simulink model "TotemPoleBoostPFCConverter"  (R2026a)
settings: Solver=ode3  StopTime=0.05  MaxStep=1e-5  AbsTol=1e-3
PreLoadFcn:
  | TotemPoleBoostPFCDefaultInputParameters;
model workspace (MAT data in the model file):
  ConverterKey = "TotemPoleBoostPFC"
undefined symbols (not defined in the file): Rload_R, totemPoleDesign, Vref
libraries: ee_lib x27, nesl_utility x23, fl_lib x12, ConverterLibrary x1
(part 1 of 3)
settings Model: Creator=vsolaise  LastModifiedBy=vsolaise
settings SimscapeCC: SimscapeNominalValues="[{\"value\":\"1\",\"unit\":\"A\"},{\"value\":\"1\",\"unit\":\"bar\"},{\"value\":\"1\",\"unit\":\"cm^2\"},{\"value\":\"1\",\"unit\":\"cm^3/s\"},{\"value\":\"1\",\"unit\":\"kJ/kg\"},{\"value\":\"1\",\"unit\":\"kW\"},{\"value\":\"1\",\"unit\":\"l\"},{\"value\":\"1\",\"unit\":\"N\"},{\"value\":\"1\",\"unit\":\"N*m\"},{\"value\":\"1\",\"unit\":\"V\"}]"  SimscapeLogDecimation=12.0  SimscapeLogDataHistory=50000.0

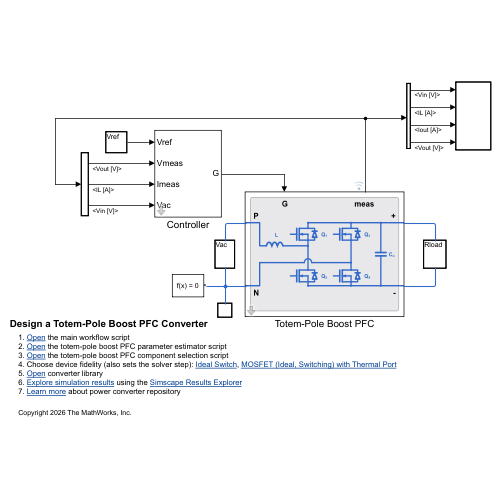
[thumbnail: Simulink's stored preview of the top-level diagram]
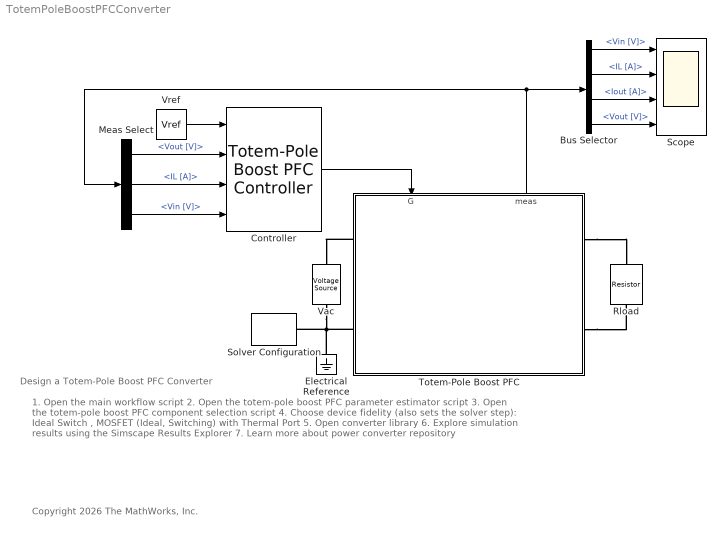
== system TotemPoleBoostPFCConverter ==
  note: Design a Totem-Pole Boost PFC Converter
  note: 1. Open the main workflow script
      | 2. Open the totem-pole boost PFC parameter estimator script
      | 3. Open the totem-pole boost PFC component selection script
      | 4. Choose device fidelity (also sets the solver step): Ideal Switch , MOSFET (Ideal, Switching) with Thermal Port
      | 5. Open converter library
      | 6. Explore simulation results using the Simscape Results Explorer
      | 7. Learn more about power converter repository
  note: Copyright 2026 The MathWorks, Inc.
  Bus Selector : BusSelector  OutputSignals=Vin [V],IL [A],Iout [A],Vout [V]
  Controller : ConverterLibrary/Controller/Power Factor Correction Converters/Totem-Pole Boost PFC Controller  outputSelect=PWM Signal  cntrlSelect=PI controller (Discrete)  VacRMS=totemPoleDesign.nomInputVoltage.value  VbaseDC=totemPoleDesign.outputVoltage.value  Pbase=totemPoleDesign.ratedPower.value  Fsw=totemPoleDesign.switchingFrequency.value  Fline=totemPoleDesign.lineFrequency.value  fastLegDeadTime=totemPoleController.fastLegDeadTime  slowLegTurnOnDelay=totemPoleController.slowLegTurnOnDelay  PrefPu=totemPoleController.PrefPu  iRefPeakMaxPu=totemPoleController.iRefPeakMaxPu  gateVoltageOn=totemPoleController.gateVoltageOn  gateVoltageOff=totemPoleController.gateVoltageOff  KpVoltage=totemPoleController.KpVoltage  KiVoltage=totemPoleController.KiVoltage  TsVoltage=totemPoleController.TsVoltage  KpCurrent=totemPoleController.KpCurrent  KiCurrent=totemPoleController.KiCurrent  dutyMax=totemPoleController.dutyMax  dutyMin=totemPoleController.dutyMin  TsCurrent=totemPoleController.TsCurrent
      link override Current Controller: LabelModeActiveChoice=PIDiscrete
      link override Gate Logic/Slow Leg Complementary PWM/Ramp Mode: LabelModeActiveChoice=FixedStep
      link override Output Mode: LabelModeActiveChoice=PWMSignal
      link override Output Mode/PWMSignal/Half Bridge PWM Generator/Ramp Mode: LabelModeActiveChoice=FixedStep
      link override Voltage Controller: LabelModeActiveChoice=PIDiscrete
      settings: SourceProductName=Simscape Power Converter Components
  Electrical Reference : fl_lib/Electrical/Electrical Elements/Electrical Reference
  Meas Select : BusSelector  OutputSignals=Vout [V],IL [A],Vin [V]
  Rload : fl_lib/Electrical/Electrical Elements/Resistor  R=Rload_R Ohm  i_specify=off  i_priority=None  i=0 A  i_nominal_specify=off  i_nominal_value=1  i_nominal_unit=A  v_specify=off  v_priority=None  v=0 V  v_nominal_specify=off  v_nominal_value=1  v_nominal_unit=V
  Scope : Scope  NumInputPorts=4
      settings: ActiveDisplayString=4  Title=Output Voltage (A)  ActiveDisplayYMinimum=393.36883974887712  ActiveDisplayYMaximum=406.39760207131951
  Solver Configuration : nesl_utility/Solver Configuration  PhysicalDomain=network_engine_domain  SubClassName=solver  LeftPortType=input  RightPortType=generic  Tones=[]  Harmonics=[]  SimulateNoise=off  Profile=off  UseLocalSampling=off  EnableSwitchedLinearOptims=on  FrequencyDomain=off  UseCCode=off  RelTol=0.001  AbsTol=0.001  MinStep=1e-09  ToWorkspace=off  RevertToSquareIcSolve=off  NumHomotopyIterations=100  PhasorMode=off  PhasorModeNumHarmonics=1  ConsistencySolver=NEWTON_XTOL_AFTER_FTOL  CanonicalOrdering=UNORDERED  OptimizeIntermediates=UNOPTIMIZED  IndexReductionMethod=DerivativeReplacement  DoDC=off  ResidualTolerance=1e-09  ConsistencyTolSource=GLOBAL  ConsistencyAbsTol=0.001  ConsistencyRelTol=0.001  ConsistencyTolFactor=0.001  UseLocalSolver=on  LocalSolverChoice=NE_BACKWARD_EULER_ADVANCER  ResolveIndetEquations=on  FunctionEvalNumThread=1  LocalSolverSampleTime=3e-7  DoFixedCost=on  MaxNonlinIter=3  MaxModeIter=2  ComputeImpulses=off  ImpulseIterations=2  LinearAlgebra=auto  LinearAlgebraNumThread=0  EquationFormulation=NE_TIME_EF  DelaysMemoryBudget=1024  AutomaticFiltering=on  FilteringTimeConstant=0.001  PartitionStorageMethod=AS_NEEDED  PartitionMemoryBudget=1024  PartitionMethod=ROBUST  MultibodyUseLocalSolver=off  MultibodyLocalSolverChoice=ODE1  MultibodyLocalSolverSampleTime=0.001
  Totem-Pole Boost PFC : Subsystem  mask(Totem-Pole Boost PFC Converter){modelOption=Simplified, ratedPower=totemPoleDesign.ratedPower.value, ratedPower_unit=W, VIn=totemPoleDesign.nomInputVoltage.value, VIn_unit=V, FRated=totemPoleDesign.lineFrequency.value, FRated_unit=Hz, VOut=totemPoleDesign.outputVoltage.value, VOut_unit=V, Fsw=totemPoleDesign.switchingFrequency.value, Fsw_unit=Hz, LBoost=totemPoleDesign.boostInductance.value, LBoost_unit=H, RLboost=totemPoleDesign.inductorESR.value, RLboost_unit=Ohm, CBoost=totemPoleDesign.outputCapacitance.value, CBoost_unit=F, Rco=totemPoleDesign.capacitorESR.value, Rco_unit=Ohm, Vco=totemPoleDesign.initialCapacitorVoltage.value, Vco_unit=V, fastLegDeviceOption=MOSFET (Ideal, Switching) with Thermal, RdsOnFast=0.04, RdsOnFast_unit=Ohm, GdsOffFast=1e-5, GdsOffFast_unit=1/Ohm, VthFast=3, VthFast_unit=V, simTempFast=25, simTempFast_unit=degC, slowLegDeviceOption=MOSFET, slowMOSFETDeviceOption=MOSFET (Ideal, Switching) with Thermal, slowDiodeDeviceOption=Ideal Diode, RdsOnSlow=0.05, RdsOnSlow_unit=Ohm, GdsOffSlow=1e-5, GdsOffSlow_unit=1/Ohm, VthSlow=3, VthSlow_unit=V, simTempSlow=25, simTempSlow_unit=degC, VfSlow=0.6, VfSlow_unit=V, RdSlow=0.01, RdSlow_unit=Ohm, GdSlow=1e-8, GdSlow_unit=1/Ohm, IhSlow=1, IhSlow_unit=A, VfFast=0.8, VfFast_unit=V, RdFast=0.001, RdFast_unit=Ohm, GdFast=1e-5, GdFast_unit=1/Ohm}
      mask prompts: modelOption "Totem-Pole Boost PFC Model Option"; ratedPower "Rated Power"; VIn "AC Input Voltage (RMS)"; FRated "Line Frequency"; VOut "DC Output Voltage"; Fsw "Switching Frequency"; LBoost "Boost Inductance"; RLboost "Inductor resistance"; CBoost "Output Capacitance"; Rco "Capacitor ESR"; Vco "Initial Output Capacitor Voltage"; fastLegDeviceOption "Fast Leg Device"; RdsOnFast "On-State Resistance"; GdsOffFast "Off-State Conductance"; VthFast "Threshold Voltage"; simTempFast "Simulation temperature"; slowLegDeviceOption "Slow Leg Device"; slowMOSFETDeviceOption "MOSFET Device"; slowDiodeDeviceOption "Diode Device"; RdsOnSlow "On-State Resistance (MOSFET)"; GdsOffSlow "Off-State Conductance"; VthSlow "Threshold Voltage"; simTempSlow "Simulation temperature"; VfSlow "Forward Voltage (Diode)"; RdSlow "On Resistance (Diode)"; GdSlow "Off Conductance (Diode)"; IhSlow "Holding current (Ih)"; VfFast "Forward Voltage (Body Diode)"; RdFast "On Resistance (Body Diode)"; GdFast "Off Conductance (Body Diode)"
      mask help: Bridgeless totem-pole boost PFC with fast and slow legs
      mask init:
      | %% Unit conversion: convert displayed values to base SI units
      | convMap = containers.Map( ...
      |     {'W','kW','MW','V','kV','mV','A','mA','F','mF','uF','nF','pF', ...
      |      'H','mH','uH','nH','Ohm','kOhm','mOhm','S','mS','1/Ohm', ...
      |      'Hz','kHz','MHz'}, ...
      |     {1, 1e3, 1e6, 1, 1e3, 1e-3, 1, 1e-3, 1, 1e-3, 1e-6, 1e-9, 1e-12, ...
      |      1, 1e-3, 1e-6, 1e-9, 1, 1e3, 1e-3, 1, 1e-3, 1, ...
      |      1, 1e3, 1e6});
      | 
      | ratedPower_SI = ratedPower * convMap(ratedPower_unit);
      | VIn_SI = VIn * convMap(VIn_unit);
      | FRated_SI = FRated * convMap(FRated_unit);
      | VOut_SI = VOut * convMap(VOut_unit);
      | Fsw_SI = Fsw * convMap(Fsw_unit);
      | LBoost_SI = LBoost * convMap(LBoost_unit);
      | RLboost_SI = RLboost * convMap(RLboost_unit);
      | CBoost_SI = CBoost * convMap(CBoost_unit);
      | Rco_SI = Rco * convMap(Rco_unit);
      | Vco_SI = Vco * convMap(Vco_unit);
      | RdsOnFast_SI = RdsOnFast * convMap(RdsOnFast_unit);
      | GdsOffFast_SI = GdsOffFast * convMap(GdsOffFast_unit);
      | VthFast_SI = VthFast * convMap(VthFast_unit);
      | VfFast_SI = VfFast * convMap(VfFast_unit);
      | RdFast_SI = RdFast * convMap(RdFast_unit);
      | GdFast_SI = GdFast * convMap(GdFast_unit);
      | RdsOnSlow_SI = RdsOnSlow * convMap(RdsOnSlow_unit);
      | GdsOffSlow_SI = GdsOffSlow * convMap(GdsOffSlow_unit);
      | VthSlow_SI = VthSlow * convMap(VthSlow_unit);
      | VfSlow_SI = VfSlow * convMap(VfSlow_unit);
      | RdSlow_SI = RdSlow * convMap(RdSlow_unit);
      | GdSlow_SI = GdSlow * convMap(GdSlow_unit);
      | IhSlow_SI = IhSlow * convMap(IhSlow_unit);
      | 
      | %% Simulation temperature (thermal MOSFET and tabulated diode)
      | % Temperature is an OFFSET unit (K = degC + 273.15), so it cannot use the
      | % multiplicative convMap; convert it explicitly. These Kelvin variables are
      | % read directly by each thermal MOSFET junction-temperature target, by each leg's
      | % Temperature Source, and by the slow-leg tabulated diodes' device simulation
      | % temperature - the only temperature input those diodes have, since they carry no
      | % thermal port.
      | if strcmp(simTempFast_unit, 'degC')
      |     simTempFast_K = simTempFast + 273.15;
      | else
      |     simTempFast_K = simTempFast;
      | end
      | if strcmp(simTempSlow_unit, 'degC')
      |     simTempSlow_K = simTempSlow + 273.15;
      | else
      |     simTempSlow_K = simTempSlow;
      | end
      | 
      | %% Apply variant selection
      | selectTotemPolePFCModelOption(gcb);
      settings: CopyFcn="set_param(gcbh,\"LinkStatus\",\"none\");"  PortSchema="{\"entries\":[{\"content\":{\"sides\":[{\"content\":{\"connectorIds\":[\"LConn1\",\"LConn2\"]},\"type\":\"ConnectorPlacement.EquallySpacedRectSide\",\"uuid\":\"1524dc94-6d10-41c3-9c4d-140b0cbad198\"},{\"content\":{\"connectorIds\":[\"RConn1\",\"RConn2\"],\"side\":\"RIGHT\"},\"type\":\"ConnectorPlacement.EquallySpacedRectSide\",\"uuid\":\"3d33c594-269c-419c-bd3b-3274925b3c44\"},{\"content\":{\"connectorIds\":[\"In1\",\"Out1\"],\"side\":\"TOP\"},\"type\":\"ConnectorPlacement.EquallySpacedRectSide\",\"uuid\":\"36540d5a-957f-45fd-8e0e-0b298bd16df8\"}]},\"type\":\"ConnectorPlacement.EquallySpacedConnector\",\"uuid\":\"4eeec72c-6b37-4cf7-b4fd-97832ebea029\"}],\"packageUris\":[\"http://schema.mathworks.com/mf0/Connector/R2020b\"],\"version\":\"1.0\"}"
      mask Help: web('TotemPoleBoostPFC.html')
      mask TypeOptions modelOption: Simplified | Detailed
      mask Callback modelOption: selectTotemPolePFCModelOption(gcb);
      mask TypeOptions ratedPower_unit: W | kW | MW
      mask TypeOptions VIn_unit: V | kV | mV
      mask TypeOptions FRated_unit: Hz | kHz
      mask TypeOptions VOut_unit: V | kV | mV
      mask TypeOptions Fsw_unit: Hz | kHz | MHz
      mask TypeOptions LBoost_unit: H | mH | uH
      mask TypeOptions RLboost_unit: Ohm | kOhm | mOhm
      mask TypeOptions CBoost_unit: F | mF | uF | nF
      mask TypeOptions Rco_unit: Ohm | kOhm | mOhm
      mask TypeOptions Vco_unit: V | kV | mV
      mask TypeOptions fastLegDeviceOption: Ideal Switch | MOSFET (Ideal, Switching) with Thermal
      mask Callback fastLegDeviceOption: selectTotemPolePFCFastLeg(gcb);
      mask TypeOptions RdsOnFast_unit: Ohm | kOhm | mOhm
      mask TypeOptions GdsOffFast_unit: 1/Ohm | S | mS
      mask TypeOptions VthFast_unit: V | kV | mV
      mask TypeOptions simTempFast_unit: degC | K
      mask TypeOptions slowLegDeviceOption: Diode | MOSFET | Thyristor
      mask Callback slowLegDeviceOption: selectTotemPolePFCSlowLeg(gcb);
      mask TypeOptions slowMOSFETDeviceOption: Ideal Switch | MOSFET (Ideal, Switching) with Thermal
      mask Callback slowMOSFETDeviceOption: selectTotemPoleSlowMOSFETDevice(gcb);
      mask TypeOptions slowDiodeDeviceOption: Ideal Diode | Tabulated Diode
      mask Callback slowDiodeDeviceOption: selectTotemPoleSlowDiodeDevice(gcb);
      mask TypeOptions RdsOnSlow_unit: Ohm | kOhm | mOhm
      mask TypeOptions GdsOffSlow_unit: 1/Ohm | S | mS
      mask TypeOptions VthSlow_unit: V | kV | mV
      mask TypeOptions simTempSlow_unit: degC | K
      mask TypeOptions VfSlow_unit: V | kV | mV
      mask TypeOptions RdSlow_unit: Ohm | kOhm | mOhm
      mask TypeOptions GdSlow_unit: 1/Ohm | S | mS
      mask TypeOptions IhSlow_unit: A
      mask TypeOptions VfFast_unit: V | kV | mV
      mask TypeOptions RdFast_unit: Ohm | kOhm | mOhm
      mask TypeOptions GdFast_unit: 1/Ohm | S | mS
      mask DialogControl Totem_PoleBoostPFCConverterParameters Prompt: Totem-Pole Boost PFC Converter Parameters
      mask DialogControl FastLegDevice Prompt: Fast Leg Device
      mask DialogControl openFastMOSFETMask Prompt: Open MOSFET block mask
      mask DialogControl openFastMOSFETMask Callback: openTotemPoleDeviceMask(gcb, 'fastThermalMOSFET');
      mask DialogControl applyFastMOSFETParam Prompt: Apply parameters to all fast leg MOSFET blocks
      mask DialogControl applyFastMOSFETParam Callback: applyTotemPoleFastMOSFETParameters(gcb);
      mask DialogControl SlowLegDevice Prompt: Slow Leg Device
      mask DialogControl openSlowMOSFETMask Prompt: Open MOSFET block mask
      mask DialogControl openSlowMOSFETMask Callback: openTotemPoleDeviceMask(gcb, 'slowThermalMOSFET');
      mask DialogControl applySlowMOSFETParam Prompt: Apply parameters to all slow leg MOSFET blocks
      mask DialogControl applySlowMOSFETParam Callback: applyTotemPoleSlowMOSFETParameters(gcb);
      mask DialogControl openSlowDiodeMask Prompt: Open Diode block mask
      mask DialogControl openSlowDiodeMask Callback: openTotemPoleDeviceMask(gcb, 'slowTabulatedDiode');
      mask DialogControl applySlowDiodeParam Prompt: Apply parameters to all slow leg Diode blocks
      mask DialogControl applySlowDiodeParam Callback: applyTotemPoleSlowDiodeParameters(gcb);
      mask DialogControl ExportPanel Prompt: Export to Unmasked Subsystem
      mask DialogControl ExportInfo Prompt: To customize the converter, export it as an unmasked subsystem with the active variant flattened - a standalone, fully-editable circuit plus a parameter file. Requires the "Variant Manager for Simulink" add-on.
      mask DialogControl exportToModel Prompt: Export
      mask DialogControl exportToModel Callback: exportConverterModelFromMask(gcb);
      mask Display:
      | slowLeg = get_param(gcb, 'slowLegDeviceOption');
      | if strcmp(slowLeg, 'Diode')
      |     image('TotemPoleDiodeIcon.svg');
      | elseif strcmp(slowLeg, 'Thyristor')
      |     image('TotemPoleThyristorIcon.svg');
      | else
      |     image('TotemPoleMOSFETIcon.svg');
      | end
  Vac : ee_lib/Sources/Voltage Source  dc_voltage=0 V  ac_voltage=VacAmp V  ac_shift=0 rad  ac_frequency=Fline Hz  noise_mode=ee.enum.sources.noise.Disabled  PSD=0 V^2/Hz  sample_time=1e-3 s  repeatability=ee.enum.sources.repeatability.NotRepeatable  user_seed=0  auto_seed=3037630589  i_specify=off  i_priority=None  i=0 A  i_nominal_specify=off  i_nominal_value=1  i_nominal_unit=A  v_specify=off  v_priority=None  v=0 V  v_nominal_specify=off  v_nominal_value=1  v_nominal_unit=V
  Vref : Constant  Value=Vref
  wires:
  Totem-Pole Boost PFC/1(meas) -> Bus Selector/1, Meas Select/1
  Vref/1 -> Controller/1
  Meas Select/1 -> Controller/2  "<Vout [V]>"
  Meas Select/2 -> Controller/3  "<IL [A]>"
  Meas Select/3 -> Controller/4  "<Vin [V]>"
  Controller/1 -> Totem-Pole Boost PFC/1(G)
  Bus Selector/1 -> Scope/1  "<Vin [V]>"
  Bus Selector/2 -> Scope/2  "<IL [A]>"
  Bus Selector/3 -> Scope/3  "<Iout [A]>"
  Bus Selector/4 -> Scope/4  "<Vout [V]>"
  connections:
  Totem-Pole Boost PFC/LConn1 -- Vac/LConn1
  Vac/RConn1 -- Electrical Reference/LConn1 -- Solver Configuration/RConn1 -- Totem-Pole Boost PFC/LConn2
  Totem-Pole Boost PFC/RConn1 -- Rload/LConn1
  Totem-Pole Boost PFC/RConn2 -- Rload/RConn1

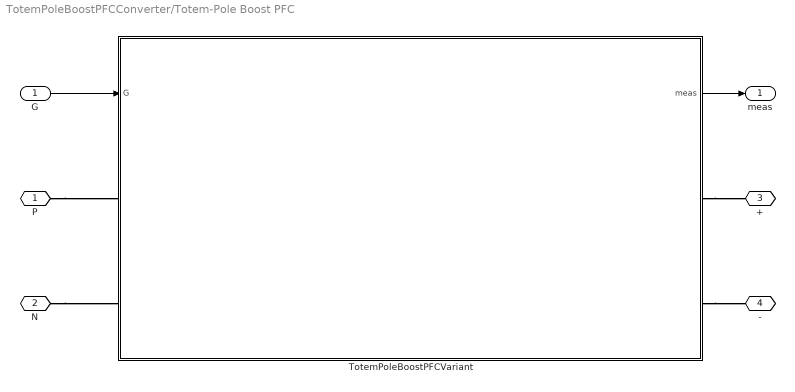
== system TotemPoleBoostPFCConverter/Totem-Pole Boost PFC ==
  G : Inport
  TotemPoleBoostPFCVariant : Subsystem  Variant=on  VariantControlMode=label  LabelModeActiveChoice=SimplifiedModel
  P : PMIOPort  Side=Left
  N : PMIOPort  Port=2  Side=Left
  + : PMIOPort  Port=3  Side=Right
  - : PMIOPort  Port=4  Side=Right
  meas : Outport
  wires:
  G/1 -> TotemPoleBoostPFCVariant/1(G)
  TotemPoleBoostPFCVariant/1(meas) -> meas/1
  connections:
  P/RConn1 -- TotemPoleBoostPFCVariant/LConn1
  N/RConn1 -- TotemPoleBoostPFCVariant/LConn2
  TotemPoleBoostPFCVariant/RConn1 -- +/RConn1
  TotemPoleBoostPFCVariant/RConn2 -- -/RConn1

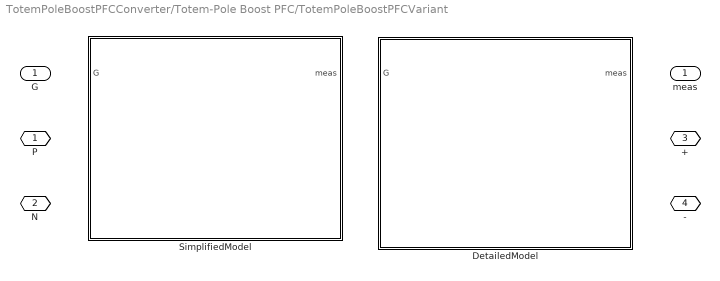
== system TotemPoleBoostPFCConverter/Totem-Pole Boost PFC/TotemPoleBoostPFCVariant ==
  G : Inport
  DetailedModel : Subsystem  VariantControl=DetailedModel
  SimplifiedModel : Subsystem  VariantControl=SimplifiedModel
  P : PMIOPort  Side=Left
  N : PMIOPort  Port=2  Side=Left
  + : PMIOPort  Port=3  Side=Right
  - : PMIOPort  Port=4  Side=Right
  meas : Outport

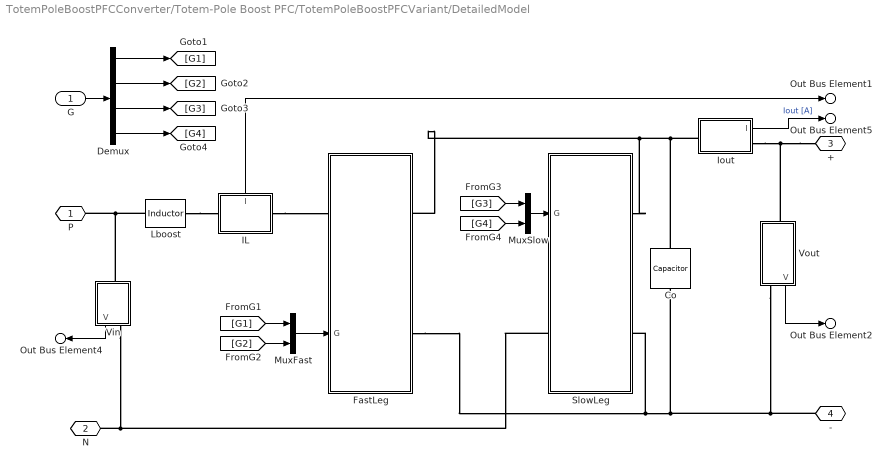
== system TotemPoleBoostPFCConverter/Totem-Pole Boost PFC/TotemPoleBoostPFCVariant/DetailedModel ==
  G : Inport
  Co : ee_lib/Passive/Capacitor  cap_option=ee.enum.passive.capacitor.capOption.const  c=CBoost_SI F  Cvec=[1e-05, 1e-06] F  Vvec=[0, 10] V  CV_table_symmetry=ee.enum.passive.capacitor.tableSymmetry.yes  f_vec=[1, 10] kHz  DFext_vec=[.8, 1.2]  enable_C_tol=ee.enum.toleranceApplication.none  averaging_period=0 s  C_tol=5  tol_distribution=ee.enum.toleranceDistribution.uniform  nSigma=4  r=Rco_SI Ohm  g=0 1/Ohm  enable_operating_limits=ee.enum.enable.no  operating_limit_action=ee.enum.passive.reportOpLim.warn  max_working_voltage_range=[-25, 25] V  power_rating=1 W  maxTemperature=85 degC  thermalEnable=false  thermalMass=1 J/K  i_specify=off  i_priority=None  i=0 A  i_nominal_specify=off  i_nominal_value=1  i_nominal_unit=A  v_specify=off  v_priority=None  v=0 V  v_nominal_specify=off  v_nominal_value=1  v_nominal_unit=V  vc_specify=on  vc_priority=High  vc=Vco_SI V  vc_nominal_specify=off  vc_nominal_value=1  vc_nominal_unit=V  T_specify=off  T_priority=None  T=298.15 K  T_nominal_specify=off  T_nominal_value=1  T_nominal_unit=K
  Demux : Demux
  FastLeg : Subsystem  Variant=on  VariantControlMode=label  LabelModeActiveChoice=SwitchingMOSFETwithThermal
      settings: PortSchema="{\"entries\":[{\"content\":{\"sides\":[{\"content\":{\"connectorIds\":[\"LConn1\",\"In1\"]},\"type\":\"ConnectorPlacement.EquallySpacedRectSide\",\"uuid\":\"77e2eceb-8f65-4ff8-b710-02732b9bb145\"},{\"content\":{\"connectorIds\":[\"RConn1\",\"RConn2\"],\"side\":\"RIGHT\"},\"type\":\"ConnectorPlacement.EquallySpacedRectSide\",\"uuid\":\"bfc7df5d-eb60-4c5b-86be-68c51cd3b8c3\"},{\"content\":{\"side\":\"TOP\"},\"type\":\"ConnectorPlacement.EquallySpacedRectSide\",\"uuid\":\"613efa33-60b7-4b5b-9311-a6c7287e5913\"}]},\"type\":\"ConnectorPlacement.EquallySpacedConnector\",\"uuid\":\"12746f96-860a-4c97-9f60-ace4c102aa63\"}],\"packageUris\":[\"http://schema.mathworks.com/mf0/Connector/R2020b\"],\"version\":\"1.0\"}"
  IL : Subsystem
      settings: PortSchema="{\"entries\":[{\"content\":{\"sides\":[{\"content\":{\"connectorIds\":[\"LConn1\"]},\"type\":\"ConnectorPlacement.EquallySpacedRectSide\",\"uuid\":\"80632e7e-66fe-49c8-894c-61cf7358e53a\"},{\"content\":{\"connectorIds\":[\"RConn1\"],\"side\":\"RIGHT\"},\"type\":\"ConnectorPlacement.EquallySpacedRectSide\",\"uuid\":\"7fb991d4-0257-47fa-8c16-238ff3f2e60c\"},{\"content\":{\"connectorIds\":[\"Out1\"],\"side\":\"TOP\"},\"type\":\"ConnectorPlacement.EquallySpacedRectSide\",\"uuid\":\"a2cf4f5e-7cb3-4577-a513-817a4fd9f07d\"}]},\"type\":\"ConnectorPlacement.EquallySpacedConnector\",\"uuid\":\"e3fac4ca-b917-4eeb-beb4-75837a4782c1\"}],\"packageUris\":[\"http://schema.mathworks.com/mf0/Connector/R2020b\"],\"version\":\"1.0\"}"
      mask Display: disp('I')
  Iout : Subsystem
      mask Display: disp('I')
  Lboost : ee_lib/Passive/Inductor  l=LBoost_SI H  enable_L_tol=ee.enum.toleranceApplication.none  L_tol=20  tol_distribution=ee.enum.toleranceDistribution.uniform  nSigma=4  r=RLboost_SI Ohm  g=1e-5 1/Ohm  enable_operating_limits=ee.enum.enable.no  operating_limit_action=ee.enum.passive.reportOpLim.warn  max_working_current=1 A  power_rating=1 W  i_L_specify=off  i_L_priority=High  i_L=0 A  i_L_nominal_specify=off  i_L_nominal_value=1  i_L_nominal_unit=A
  MuxFast : Mux  Inputs=2
  MuxSlow : Mux  Inputs=2
  SlowLeg : Subsystem  Variant=on  VariantControlMode=label  LabelModeActiveChoice=MOSFET
  Vin : Subsystem
      mask Display: disp('V')
  Vout : Subsystem
      settings: PortSchema="{\"entries\":[{\"content\":{\"sides\":[{\"content\":{\"connectorIds\":[\"LConn1\"]},\"type\":\"ConnectorPlacement.EquallySpacedRectSide\",\"uuid\":\"80632e7e-66fe-49c8-894c-61cf7358e53a\"},{\"content\":{\"connectorIds\":[\"RConn1\",\"Out1\"],\"side\":\"RIGHT\"},\"type\":\"ConnectorPlacement.EquallySpacedRectSide\",\"uuid\":\"7fb991d4-0257-47fa-8c16-238ff3f2e60c\"},{\"content\":{\"side\":\"TOP\"},\"type\":\"ConnectorPlacement.EquallySpacedRectSide\",\"uuid\":\"a2cf4f5e-7cb3-4577-a513-817a4fd9f07d\"}]},\"type\":\"ConnectorPlacement.EquallySpacedConnector\",\"uuid\":\"e3fac4ca-b917-4eeb-beb4-75837a4782c1\"}],\"packageUris\":[\"http://schema.mathworks.com/mf0/Connector/R2020b\"],\"version\":\"1.0\"}"
      mask Display: disp('V')
  P : PMIOPort  Side=Left
  N : PMIOPort  Port=2  Side=Left
  + : PMIOPort  Port=3  Side=Right
  - : PMIOPort  Port=4  Side=Right
  Out Bus Element1 : Outport  PortName=meas  Element=IL [A]
  Out Bus Element2 : Outport  PortName=meas  Element=Vout [V]
  Out Bus Element4 : Outport  PortName=meas  Element=Vin [V]
  Out Bus Element5 : Outport  PortName=meas  Element=Iout [A]
  wires:
  G/1 -> Demux/1
  Demux/4 -> [G4]
  Demux/3 -> [G3]
  Demux/2 -> [G2]
  Demux/1 -> [G1]
  Vout/1(V) -> Out Bus Element2/1
  Iout/1(I) -> Out Bus Element5/1  "Iout [A]"
  IL/1(I) -> Out Bus Element1/1
  [G4] -> MuxSlow/2
  [G3] -> MuxSlow/1
  MuxSlow/1 -> SlowLeg/1(G)
  Vin/1(V) -> Out Bus Element4/1
  [G2] -> MuxFast/2
  [G1] -> MuxFast/1
  MuxFast/1 -> FastLeg/1(G)
  connections:
  Vout/RConn1 -- -/RConn1 -- Co/RConn1 -- FastLeg/RConn2 -- SlowLeg/RConn2
  IL/RConn1 -- FastLeg/LConn1
  +/RConn1 -- Vout/LConn1 -- Iout/RConn1
  N/RConn1 -- SlowLeg/LConn1 -- Vin/RConn1
  Lboost/RConn1 -- IL/LConn1
  Iout/LConn1 -- Co/LConn1 -- FastLeg/RConn1 -- SlowLeg/RConn1
  Vin/LConn1 -- P/RConn1 -- Lboost/LConn1

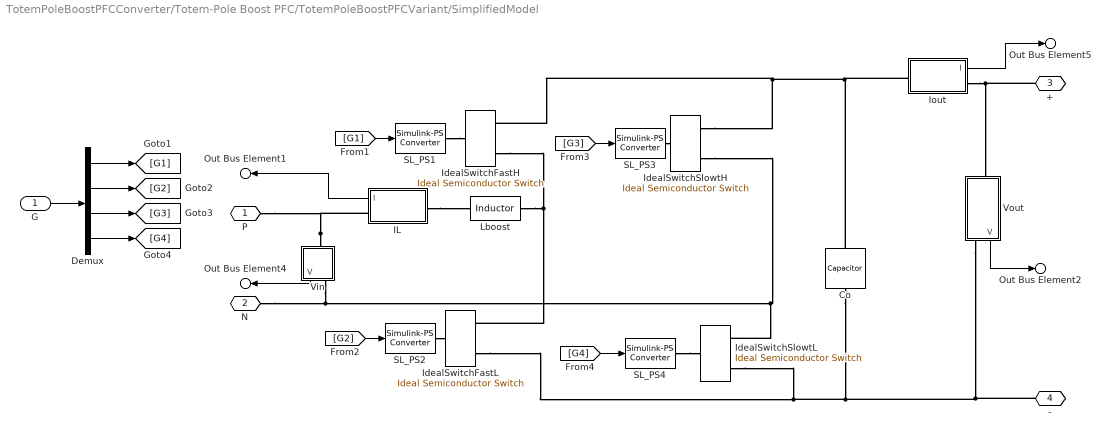
== system TotemPoleBoostPFCConverter/Totem-Pole Boost PFC/TotemPoleBoostPFCVariant/SimplifiedModel ==
  G : Inport
  Co : ee_lib/Passive/Capacitor  cap_option=ee.enum.passive.capacitor.capOption.const  c=CBoost_SI F  Cvec=[1e-05, 1e-06] F  Vvec=[0, 10] V  CV_table_symmetry=ee.enum.passive.capacitor.tableSymmetry.yes  f_vec=[1, 10] kHz  DFext_vec=[.8, 1.2]  enable_C_tol=ee.enum.toleranceApplication.none  averaging_period=0 s  C_tol=5  tol_distribution=ee.enum.toleranceDistribution.uniform  nSigma=4  r=Rco_SI Ohm  g=0 1/Ohm  enable_operating_limits=ee.enum.enable.no  operating_limit_action=ee.enum.passive.reportOpLim.warn  max_working_voltage_range=[-25, 25] V  power_rating=1 W  maxTemperature=85 degC  thermalEnable=false  thermalMass=1 J/K  i_specify=off  i_priority=None  i=0 A  i_nominal_specify=off  i_nominal_value=1  i_nominal_unit=A  v_specify=off  v_priority=None  v=0 V  v_nominal_specify=off  v_nominal_value=1  v_nominal_unit=V  vc_specify=on  vc_priority=High  vc=Vco_SI V  vc_nominal_specify=off  vc_nominal_value=1  vc_nominal_unit=V  T_specify=off  T_priority=None  T=298.15 K  T_nominal_specify=off  T_nominal_value=1  T_nominal_unit=K
  Demux : Demux
  IL : Subsystem
      settings: PortSchema="{\"entries\":[{\"content\":{\"sides\":[{\"content\":{\"connectorIds\":[\"Out1\",\"LConn1\"]},\"type\":\"ConnectorPlacement.EquallySpacedRectSide\",\"uuid\":\"39b7e526-9a68-4c73-9ad6-fd149fea363a\"},{\"content\":{\"connectorIds\":[\"RConn1\"],\"side\":\"RIGHT\"},\"type\":\"ConnectorPlacement.EquallySpacedRectSide\",\"uuid\":\"ee3f62d2-02c4-4290-ad83-c24a9e891d89\"},{\"content\":{\"side\":\"TOP\"},\"type\":\"ConnectorPlacement.EquallySpacedRectSide\",\"uuid\":\"a8618696-d9d3-41f8-b97f-996b903ae337\"}]},\"type\":\"ConnectorPlacement.EquallySpacedConnector\",\"uuid\":\"57ec1f0b-c67f-47bc-9e24-5102208e6cfb\"}],\"packageUris\":[\"http://schema.mathworks.com/mf0/Connector/R2020b\"],\"version\":\"1.0\"}"
      mask Display: disp('I')
  IdealSwitchFastH : ee_lib/Semiconductors & Converters/Ideal Semiconductor Switch  port_option=ee.enum.controlport.ps  Ron=RdsOnFast_SI Ohm  Goff=GdsOffFast_SI 1/Ohm  Vth=VthFast_SI V  diode_param=ee.enum.semiconductors.protectionDiode.nodynamics  diode_Vf=VfFast_SI V  diode_Ron=RdFast_SI Ohm  diode_Goff=GdFast_SI 1/Ohm  diode_C=50e-9 F  diode_iRM=-235 A  diode_iF=300 A  diode_idot=-50 A/us  diode_trr_param=ee.enum.converters.diodetrr.trr_factor  diode_trr_factor=3  diode_trr=15 us  diode_Qrr=1500 s*uA
  IdealSwitchFastL : ee_lib/Semiconductors & Converters/Ideal Semiconductor Switch  port_option=ee.enum.controlport.ps  Ron=RdsOnFast_SI Ohm  Goff=GdsOffFast_SI 1/Ohm  Vth=VthFast_SI V  diode_param=ee.enum.semiconductors.protectionDiode.nodynamics  diode_Vf=VfFast_SI V  diode_Ron=RdFast_SI Ohm  diode_Goff=GdFast_SI 1/Ohm  diode_C=50e-9 F  diode_iRM=-235 A  diode_iF=300 A  diode_idot=-50 A/us  diode_trr_param=ee.enum.converters.diodetrr.trr_factor  diode_trr_factor=3  diode_trr=15 us  diode_Qrr=1500 s*uA
  IdealSwitchSlowtH : ee_lib/Semiconductors & Converters/Ideal Semiconductor Switch  port_option=ee.enum.controlport.ps  Ron=RdsOnSlow_SI Ohm  Goff=GdsOffSlow_SI 1/Ohm  Vth=VthSlow_SI V  diode_param=ee.enum.semiconductors.protectionDiode.nodynamics  diode_Vf=VfSlow_SI V  diode_Ron=RdSlow_SI Ohm  diode_Goff=GdSlow_SI 1/Ohm  diode_C=50e-9 F  diode_iRM=-235 A  diode_iF=300 A  diode_idot=-50 A/us  diode_trr_param=ee.enum.converters.diodetrr.trr_factor  diode_trr_factor=3  diode_trr=15 us  diode_Qrr=1500 s*uA
  IdealSwitchSlowtL : ee_lib/Semiconductors & Converters/Ideal Semiconductor Switch  port_option=ee.enum.controlport.ps  Ron=RdsOnSlow_SI Ohm  Goff=GdsOffSlow_SI 1/Ohm  Vth=VthSlow_SI V  diode_param=ee.enum.semiconductors.protectionDiode.nodynamics  diode_Vf=VfSlow_SI V  diode_Ron=RdSlow_SI Ohm  diode_Goff=GdSlow_SI 1/Ohm  diode_C=50e-9 F  diode_iRM=-235 A  diode_iF=300 A  diode_idot=-50 A/us  diode_trr_param=ee.enum.converters.diodetrr.trr_factor  diode_trr_factor=3  diode_trr=15 us  diode_Qrr=1500 s*uA
  Iout : Subsystem
      mask Display: disp('I')
  Lboost : ee_lib/Passive/Inductor  l=LBoost_SI H  enable_L_tol=ee.enum.toleranceApplication.none  L_tol=20  tol_distribution=ee.enum.toleranceDistribution.uniform  nSigma=4  r=RLboost_SI Ohm  g=1e-5 1/Ohm  enable_operating_limits=ee.enum.enable.no  operating_limit_action=ee.enum.passive.reportOpLim.warn  max_working_current=1 A  power_rating=1 W  i_L_specify=off  i_L_priority=High  i_L=0 A  i_L_nominal_specify=off  i_L_nominal_value=1  i_L_nominal_unit=A
  SL_PS{1..4} (4 alike) : nesl_utility/Simulink-PS Converter  PhysicalDomain=network_engine_domain  SubClassName=ps_input  LeftPortType=input  RightPortType=output  PseudoPeriodic=off  Frequencies=[]  NoiseDistribution=none  NoiseParameters=[]  Unit=1  AffineConversion=off  FilteringAndDerivatives=provide  SimscapeFilterOrder=1  InputFilterTimeConstant=0.001  UdotUserProvided=0
  Vin : Subsystem
      mask Display: disp('V')
  Vout : Subsystem
      settings: PortSchema="{\"entries\":[{\"content\":{\"sides\":[{\"content\":{\"connectorIds\":[\"LConn1\"]},\"type\":\"ConnectorPlacement.EquallySpacedRectSide\",\"uuid\":\"39b7e526-9a68-4c73-9ad6-fd149fea363a\"},{\"content\":{\"connectorIds\":[\"RConn1\",\"Out1\"],\"side\":\"RIGHT\"},\"type\":\"ConnectorPlacement.EquallySpacedRectSide\",\"uuid\":\"ee3f62d2-02c4-4290-ad83-c24a9e891d89\"},{\"content\":{\"side\":\"TOP\"},\"type\":\"ConnectorPlacement.EquallySpacedRectSide\",\"uuid\":\"a8618696-d9d3-41f8-b97f-996b903ae337\"}]},\"type\":\"ConnectorPlacement.EquallySpacedConnector\",\"uuid\":\"57ec1f0b-c67f-47bc-9e24-5102208e6cfb\"}],\"packageUris\":[\"http://schema.mathworks.com/mf0/Connector/R2020b\"],\"version\":\"1.0\"}"
      mask Display: disp('V')
  P : PMIOPort  Side=Left
  N : PMIOPort  Port=2  Side=Left
  + : PMIOPort  Port=3  Side=Right
  - : PMIOPort  Port=4  Side=Right
  Out Bus Element1 : Outport  PortName=meas  Element=IL [A]
  Out Bus Element2 : Outport  PortName=meas  Element=Vout [V]
  Out Bus Element4 : Outport  PortName=meas  Element=Vin [V]
  Out Bus Element5 : Outport  PortName=meas  Element=Iout [A]
  wires:
  Iout/1(I) -> Out Bus Element5/1
  Vin/1(V) -> Out Bus Element4/1
  Vout/1(V) -> Out Bus Element2/1
  IL/1(I) -> Out Bus Element1/1
  [G4] -> SL_PS4/1
  [G3] -> SL_PS3/1
  [G2] -> SL_PS2/1
  [G1] -> SL_PS1/1
  Demux/4 -> [G4]
  Demux/3 -> [G3]
  Demux/2 -> [G2]
  Demux/1 -> [G1]
  G/1 -> Demux/1
  connections:
  Vin/RConn1 -- N/RConn1 -- IdealSwitchSlowtH/RConn2 -- IdealSwitchSlowtL/RConn1
  SL_PS4/RConn1 -- IdealSwitchSlowtL/LConn1
  SL_PS3/RConn1 -- IdealSwitchSlowtH/LConn1
  Co/LConn1 -- Iout/LConn1 -- IdealSwitchSlowtH/RConn1 -- IdealSwitchFastH/RConn1
  IL/RConn1 -- Lboost/LConn1
  +/RConn1 -- Vout/LConn1 -- Iout/RConn1
  -/RConn1 -- Vout/RConn1 -- Co/RConn1 -- IdealSwitchSlowtL/RConn2 -- IdealSwitchFastL/RConn2
  Vin/LConn1 -- P/RConn1 -- IL/LConn1
  SL_PS2/RConn1 -- IdealSwitchFastL/LConn1
  SL_PS1/RConn1 -- IdealSwitchFastH/LConn1
  IdealSwitchFastH/RConn2 -- IdealSwitchFastL/RConn1 -- Lboost/RConn1

== system TotemPoleBoostPFCConverter/Totem-Pole Boost PFC/TotemPoleBoostPFCVariant/DetailedModel/FastLeg ==
  G : Inport
  IdealSwitch : Subsystem  VariantControl=IdealSwitch
  SwitchingMOSFETwithThermal : Subsystem  VariantControl=SwitchingMOSFETwithThermal
  Mid : PMIOPort  Side=Left
  DC+ : PMIOPort  Port=2  Side=Right
  DC- : PMIOPort  Port=3  Side=Right

== system TotemPoleBoostPFCConverter/Totem-Pole Boost PFC/TotemPoleBoostPFCVariant/DetailedModel/IL ==
  Current Sensor : fl_lib/Electrical/Electrical Sensors/Current Sensor
  PS-Simulink Converter : nesl_utility/PS-Simulink Converter  PhysicalDomain=network_engine_domain  SubClassName=ps_output  LeftPortType=input  RightPortType=output  PseudoPeriodic=off  Frequencies=[]  VectorFormat=inherit  Unit=inherit  AffineConversion=off
  + : PMIOPort  Side=Left
  - : PMIOPort  Port=2  Side=Right
  I : Outport
  wires:
  PS-Simulink Converter/1 -> I/1
  connections:
  +/RConn1 -- Current Sensor/LConn1
  Current Sensor/RConn2 -- -/RConn1
  Current Sensor/RConn1 -- PS-Simulink Converter/LConn1

== system TotemPoleBoostPFCConverter/Totem-Pole Boost PFC/TotemPoleBoostPFCVariant/DetailedModel/Iout ==
  Current Sensor : fl_lib/Electrical/Electrical Sensors/Current Sensor
  PS-Simulink Converter : nesl_utility/PS-Simulink Converter  PhysicalDomain=network_engine_domain  SubClassName=ps_output  LeftPortType=input  RightPortType=output  PseudoPeriodic=off  Frequencies=[]  VectorFormat=inherit  Unit=inherit  AffineConversion=off
  + : PMIOPort  Side=Left
  - : PMIOPort  Port=2  Side=Right
  I : Outport
  wires:
  PS-Simulink Converter/1 -> I/1
  connections:
  +/RConn1 -- Current Sensor/LConn1
  Current Sensor/RConn2 -- -/RConn1
  Current Sensor/RConn1 -- PS-Simulink Converter/LConn1

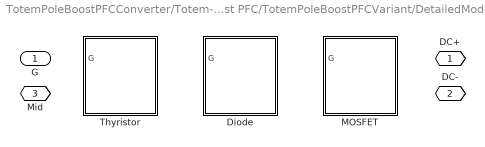
== system TotemPoleBoostPFCConverter/Totem-Pole Boost PFC/TotemPoleBoostPFCVariant/DetailedModel/SlowLeg ==
  G : Inport
  Diode : Subsystem  Variant=on  VariantControlMode=label  VariantControl=Diode  LabelModeActiveChoice=IdealDiode
  MOSFET : Subsystem  Variant=on  VariantControlMode=label  VariantControl=MOSFET  LabelModeActiveChoice=SwitchingMOSFETwithThermal
  Thyristor : Subsystem  VariantControl=Thyristor
  DC+ : PMIOPort  Side=Right
  DC- : PMIOPort  Port=2  Side=Right
  Mid : PMIOPort  Port=3  Side=Left

== system TotemPoleBoostPFCConverter/Totem-Pole Boost PFC/TotemPoleBoostPFCVariant/DetailedModel/Vin ==
  PS-Simulink Converter : nesl_utility/PS-Simulink Converter  PhysicalDomain=network_engine_domain  SubClassName=ps_output  LeftPortType=input  RightPortType=output  PseudoPeriodic=off  Frequencies=[]  VectorFormat=inherit  Unit=inherit  AffineConversion=off
  Voltage Sensor : fl_lib/Electrical/Electrical Sensors/Voltage Sensor
  + : PMIOPort  Side=Left
  - : PMIOPort  Port=2  Side=Right
  V : Outport
  wires:
  PS-Simulink Converter/1 -> V/1
  connections:
  +/RConn1 -- Voltage Sensor/LConn1
  Voltage Sensor/RConn2 -- -/RConn1
  Voltage Sensor/RConn1 -- PS-Simulink Converter/LConn1

== system TotemPoleBoostPFCConverter/Totem-Pole Boost PFC/TotemPoleBoostPFCVariant/DetailedModel/Vout ==
  PS-Simulink Converter : nesl_utility/PS-Simulink Converter  PhysicalDomain=network_engine_domain  SubClassName=ps_output  LeftPortType=input  RightPortType=output  PseudoPeriodic=off  Frequencies=[]  VectorFormat=inherit  Unit=inherit  AffineConversion=off
  Voltage Sensor : fl_lib/Electrical/Electrical Sensors/Voltage Sensor
  + : PMIOPort  Side=Left
  - : PMIOPort  Port=2  Side=Right
  V : Outport
  wires:
  PS-Simulink Converter/1 -> V/1
  connections:
  +/RConn1 -- Voltage Sensor/LConn1
  Voltage Sensor/RConn2 -- -/RConn1
  Voltage Sensor/RConn1 -- PS-Simulink Converter/LConn1

== system TotemPoleBoostPFCConverter/Totem-Pole Boost PFC/TotemPoleBoostPFCVariant/SimplifiedModel/IL ==
  Current Sensor : fl_lib/Electrical/Electrical Sensors/Current Sensor
  PS-Simulink Converter : nesl_utility/PS-Simulink Converter  PhysicalDomain=network_engine_domain  SubClassName=ps_output  LeftPortType=input  RightPortType=output  PseudoPeriodic=off  Frequencies=[]  VectorFormat=inherit  Unit=inherit  AffineConversion=off
  + : PMIOPort  Side=Left
  - : PMIOPort  Port=2  Side=Right
  I : Outport
  wires:
  PS-Simulink Converter/1 -> I/1
  connections:
  +/RConn1 -- Current Sensor/LConn1
  Current Sensor/RConn2 -- -/RConn1
  Current Sensor/RConn1 -- PS-Simulink Converter/LConn1

== system TotemPoleBoostPFCConverter/Totem-Pole Boost PFC/TotemPoleBoostPFCVariant/SimplifiedModel/Iout ==
  Current Sensor : fl_lib/Electrical/Electrical Sensors/Current Sensor
  PS-Simulink Converter : nesl_utility/PS-Simulink Converter  PhysicalDomain=network_engine_domain  SubClassName=ps_output  LeftPortType=input  RightPortType=output  PseudoPeriodic=off  Frequencies=[]  VectorFormat=inherit  Unit=inherit  AffineConversion=off
  + : PMIOPort  Side=Left
  - : PMIOPort  Port=2  Side=Right
  I : Outport
  wires:
  PS-Simulink Converter/1 -> I/1
  connections:
  +/RConn1 -- Current Sensor/LConn1
  Current Sensor/RConn2 -- -/RConn1
  Current Sensor/RConn1 -- PS-Simulink Converter/LConn1

== system TotemPoleBoostPFCConverter/Totem-Pole Boost PFC/TotemPoleBoostPFCVariant/SimplifiedModel/Vin ==
  PS-Simulink Converter : nesl_utility/PS-Simulink Converter  PhysicalDomain=network_engine_domain  SubClassName=ps_output  LeftPortType=input  RightPortType=output  PseudoPeriodic=off  Frequencies=[]  VectorFormat=inherit  Unit=inherit  AffineConversion=off
  Voltage Sensor : fl_lib/Electrical/Electrical Sensors/Voltage Sensor
  + : PMIOPort  Side=Left
  - : PMIOPort  Port=2  Side=Right
  V : Outport
  wires:
  PS-Simulink Converter/1 -> V/1
  connections:
  +/RConn1 -- Voltage Sensor/LConn1
  Voltage Sensor/RConn2 -- -/RConn1
  Voltage Sensor/RConn1 -- PS-Simulink Converter/LConn1

== system TotemPoleBoostPFCConverter/Totem-Pole Boost PFC/TotemPoleBoostPFCVariant/SimplifiedModel/Vout ==
  PS-Simulink Converter : nesl_utility/PS-Simulink Converter  PhysicalDomain=network_engine_domain  SubClassName=ps_output  LeftPortType=input  RightPortType=output  PseudoPeriodic=off  Frequencies=[]  VectorFormat=inherit  Unit=inherit  AffineConversion=off
  Voltage Sensor : fl_lib/Electrical/Electrical Sensors/Voltage Sensor
  + : PMIOPort  Side=Left
  - : PMIOPort  Port=2  Side=Right
  V : Outport
  wires:
  PS-Simulink Converter/1 -> V/1
  connections:
  +/RConn1 -- Voltage Sensor/LConn1
  Voltage Sensor/RConn2 -- -/RConn1
  Voltage Sensor/RConn1 -- PS-Simulink Converter/LConn1

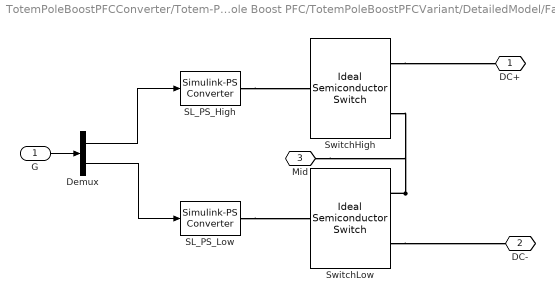
== system TotemPoleBoostPFCConverter/Totem-Pole Boost PFC/TotemPoleBoostPFCVariant/DetailedModel/FastLeg/IdealSwitch ==
  G : Inport
  Demux : Demux  Outputs=2
  SL_PS_High : nesl_utility/Simulink-PS Converter  PhysicalDomain=network_engine_domain  SubClassName=ps_input  LeftPortType=input  RightPortType=output  PseudoPeriodic=off  Frequencies=[]  NoiseDistribution=none  NoiseParameters=[]  Unit=1  AffineConversion=off  FilteringAndDerivatives=provide  SimscapeFilterOrder=1  InputFilterTimeConstant=0.001  UdotUserProvided=0
  SL_PS_Low : nesl_utility/Simulink-PS Converter  PhysicalDomain=network_engine_domain  SubClassName=ps_input  LeftPortType=input  RightPortType=output  PseudoPeriodic=off  Frequencies=[]  NoiseDistribution=none  NoiseParameters=[]  Unit=1  AffineConversion=off  FilteringAndDerivatives=provide  SimscapeFilterOrder=1  InputFilterTimeConstant=0.001  UdotUserProvided=0
  SwitchHigh : ee_lib/Semiconductors & Converters/Ideal Semiconductor Switch  port_option=ee.enum.controlport.ps  Ron=RdsOnFast_SI Ohm  Goff=GdsOffFast_SI 1/Ohm  Vth=VthFast_SI V  diode_param=ee.enum.semiconductors.protectionDiode.nodynamics  diode_Vf=VfFast_SI V  diode_Ron=RdFast_SI Ohm  diode_Goff=GdFast_SI 1/Ohm  diode_C=50e-9 F  diode_iRM=-235 A  diode_iF=300 A  diode_idot=-50 A/us  diode_trr_param=ee.enum.converters.diodetrr.trr_factor  diode_trr_factor=3  diode_trr=15 us  diode_Qrr=1500 s*uA
  SwitchLow : ee_lib/Semiconductors & Converters/Ideal Semiconductor Switch  port_option=ee.enum.controlport.ps  Ron=RdsOnFast_SI Ohm  Goff=GdsOffFast_SI 1/Ohm  Vth=VthFast_SI V  diode_param=ee.enum.semiconductors.protectionDiode.nodynamics  diode_Vf=VfFast_SI V  diode_Ron=RdFast_SI Ohm  diode_Goff=GdFast_SI 1/Ohm  diode_C=50e-9 F  diode_iRM=-235 A  diode_iF=300 A  diode_idot=-50 A/us  diode_trr_param=ee.enum.converters.diodetrr.trr_factor  diode_trr_factor=3  diode_trr=15 us  diode_Qrr=1500 s*uA
  DC+ : PMIOPort  Side=Right
  DC- : PMIOPort  Port=2  Side=Right
  Mid : PMIOPort  Port=3  Side=Left
  wires:
  G/1 -> Demux/1
  Demux/1 -> SL_PS_High/1
  Demux/2 -> SL_PS_Low/1
  connections:
  SL_PS_Low/RConn1 -- SwitchLow/LConn1
  SL_PS_High/RConn1 -- SwitchHigh/LConn1
  SwitchLow/RConn2 -- DC-/RConn1
  SwitchLow/RConn1 -- Mid/RConn1 -- SwitchHigh/RConn2
  SwitchHigh/RConn1 -- DC+/RConn1
